simulink model "converttype"  (R2023a)
settings: Solver=VariableStepAuto  StartTime=0.0  StopTime=10.0  RelTol=1e-3
settings Model: Creator=zqinghua  LastModifiedBy=zqinghua

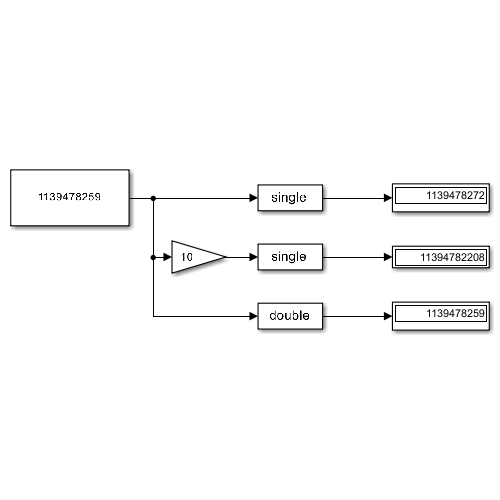
[thumbnail: Simulink's stored preview of the top-level diagram]
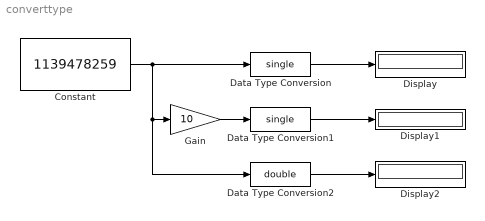
== system converttype ==
  Constant : Constant  Value=1139478259  OutDataTypeStr=uint32
  Data Type Conversion : DataTypeConversion  OutDataTypeStr=single  SaturateOnIntegerOverflow=off  RndMeth=Floor
  Data Type Conversion1 : DataTypeConversion  OutDataTypeStr=single  SaturateOnIntegerOverflow=off  RndMeth=Floor
  Data Type Conversion2 : DataTypeConversion  OutDataTypeStr=double  SaturateOnIntegerOverflow=off  RndMeth=Floor
  Display : Display
      settings: Format=decimal (Stored Integer)
  Display1 : Display
      settings: Format=decimal (Stored Integer)
  Display2 : Display
      settings: Format=decimal (Stored Integer)
  Gain : Gain  Gain=10
  wires:
  Constant/1 -> Data Type Conversion2/1, Gain/1, Data Type Conversion/1
  Gain/1 -> Data Type Conversion1/1
  Data Type Conversion/1 -> Display/1
  Data Type Conversion1/1 -> Display1/1
  Data Type Conversion2/1 -> Display2/1
